simulink model "ElectricThrottleControl"  (R2024b)
settings: Solver=VariableStepAuto  StartTime=0.0  StopTime=0.5  RelTol=1e-3
settings Model: DataDictionary=SysMLArchModel_DD.sldd  Creator=ykamatan  LastModifiedBy=ykamatan
settings DataIOCC: ExternalInput=Scenario.getElement(1),Scenario.getElement(2),Scenario.getElement(3),Scenario.getElement(4)  LoadExternalInput=on

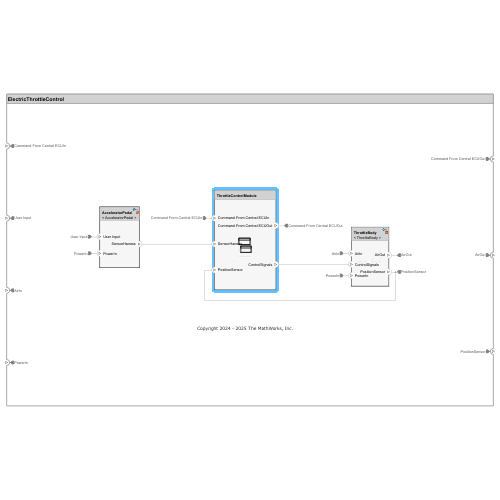
[thumbnail: Simulink's stored preview of the top-level diagram]
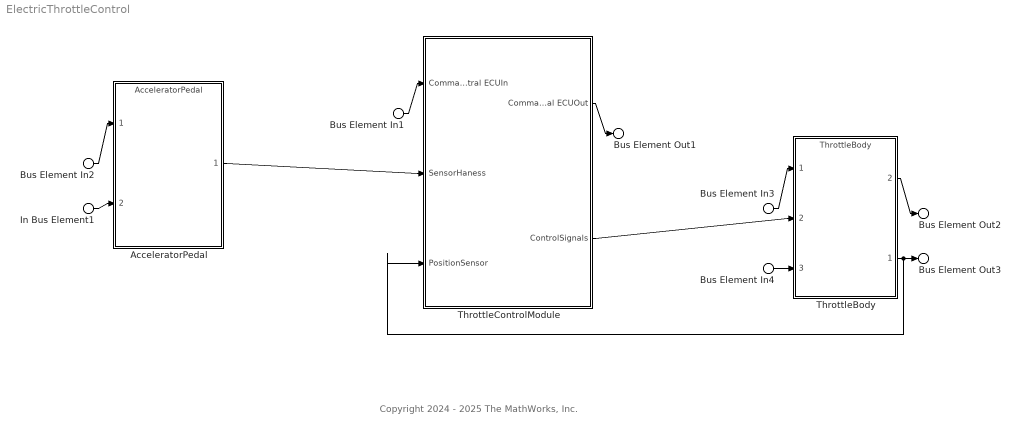
== system ElectricThrottleControl ==
  note: Copyright 2024 - 2025 The MathWorks, Inc.
  Bus Element In1 : Inport  PortName=Command From Central ECUIn
  Bus Element In2 : Inport  Port=2  PortName=User Input
  Bus Element In3 : Inport  Port=3  PortName=AirIn
  Bus Element In4 : Inport  Port=4  PortName=PowerIn
  In Bus Element1 : Inport  Port=4  PortName=PowerIn
  AcceleratorPedal : ModelReference  ModelNameDialog=AcceleratorPedal  SimulationMode=Normal  ModelReferenceVersion=1.6
      settings: PortSchema="{\"entries\":[{\"content\":{\"headerSize\":38,\"margin\":15,\"minimumSpacing\":25,\"sides\":[{\"content\":{\"connectorIds\":[\"In1\",\"In2\"]},\"type\":\"ConnectorPlacement.EquallySpacedRectSide\",\"uuid\":\"1abb2ddf-551e-4f22-91e6-e0600bbcfdfe\"},{\"content\":{\"connectorIds\":[\"Out1\"],\"side\":\"RIGHT\"},\"type\":\"ConnectorPlacement.EquallySpacedRectSide\",\"uuid\":\"67bebb00-cc4b-4347-b86c-01c9aefb7a18\"},{\"content\":{\"side\":\"TOP\"},\"type\":\"ConnectorPlacement.EquallySpacedRectSide\",\"uuid\":\"4c338e4e-b99e-491b-b4b2-5dc7867eebc8\"}]},\"type\":\"ConnectorPlacement.EquallySpacedConnector\",\"uuid\":\"67761126-1f2c-45f7-9918-87ef92113f7f\"}],\"packageUris\":[\"http://schema.mathworks.com/mf0/Connector/R2020b\"],\"version\":\"1.0\"}"
  ThrottleBody : ModelReference  ModelNameDialog=ThrottleBody  UsingDefaultArgumentValue=0,0,0,0,0,0,0  SimulationMode=Normal  ModelReferenceVersion=2.0
      settings: PortSchema="{\"entries\":[{\"content\":{\"headerSize\":38,\"margin\":15,\"minimumSpacing\":25,\"sides\":[{\"content\":{\"connectorIds\":[\"In1\",\"In2\",\"In3\"]},\"type\":\"ConnectorPlacement.EquallySpacedRectSide\",\"uuid\":\"1abb2ddf-551e-4f22-91e6-e0600bbcfdfe\"},{\"content\":{\"connectorIds\":[\"Out2\",\"Out1\"],\"side\":\"RIGHT\"},\"type\":\"ConnectorPlacement.EquallySpacedRectSide\",\"uuid\":\"67bebb00-cc4b-4347-b86c-01c9aefb7a18\"},{\"content\":{\"side\":\"TOP\"},\"type\":\"ConnectorPlacement.EquallySpacedRectSide\",\"uuid\":\"4c338e4e-b99e-491b-b4b2-5dc7867eebc8\"}]},\"type\":\"ConnectorPlacement.EquallySpacedConnector\",\"uuid\":\"67761126-1f2c-45f7-9918-87ef92113f7f\"}],\"packageUris\":[\"http://schema.mathworks.com/mf0/Connector/R2020b\"],\"version\":\"1.0\"}"
  ThrottleControlModule : Subsystem
      settings: PortSchema="{\"entries\":[{\"content\":{\"headerSize\":26,\"margin\":15,\"minimumSpacing\":25,\"sides\":[{\"content\":{\"connectorIds\":[\"In1\",\"In2\",\"In3\"]},\"type\":\"ConnectorPlacement.EquallySpacedRectSide\",\"uuid\":\"1abb2ddf-551e-4f22-91e6-e0600bbcfdfe\"},{\"content\":{\"connectorIds\":[\"Out1\",\"Out2\"],\"side\":\"RIGHT\"},\"type\":\"ConnectorPlacement.EquallySpacedRectSide\",\"uuid\":\"67bebb00-cc4b-4347-b86c-01c9aefb7a18\"},{\"content\":{\"side\":\"TOP\"},\"type\":\"ConnectorPlacement.EquallySpacedRectSide\",\"uuid\":\"4c338e4e-b99e-491b-b4b2-5dc7867eebc8\"}]},\"type\":\"ConnectorPlacement.EquallySpacedConnector\",\"uuid\":\"67761126-1f2c-45f7-9918-87ef92113f7f\"}],\"packageUris\":[\"http://schema.mathworks.com/mf0/Connector/R2020b\"],\"version\":\"1.0\"}"
  Bus Element Out1 : Outport  PortName=Command From Central ECUOut
  Bus Element Out2 : Outport  Port=2  PortName=AirOut
  Bus Element Out3 : Outport  Port=3  PortName=PositionSensor
  wires:
  Bus Element In1/1 -> ThrottleControlModule/1(Command From Central ECUIn)
  ThrottleControlModule/1(Command From Central ECUOut) -> Bus Element Out1/1
  In Bus Element1/1 -> AcceleratorPedal/2
  Bus Element In2/1 -> AcceleratorPedal/1
  AcceleratorPedal/1 -> ThrottleControlModule/2(SensorHaness)
  Bus Element In3/1 -> ThrottleBody/1
  ThrottleControlModule/2(ControlSignals) -> ThrottleBody/2
  Bus Element In4/1 -> ThrottleBody/3
  ThrottleBody/2 -> Bus Element Out2/1
  ThrottleBody/1 -> ThrottleControlModule/3(PositionSensor), Bus Element Out3/1

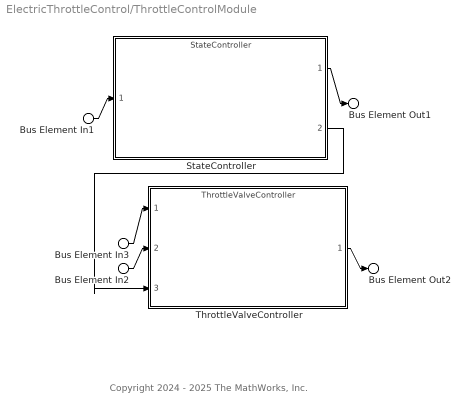
== system ElectricThrottleControl/ThrottleControlModule ==
  note: Copyright 2024 - 2025 The MathWorks, Inc.
  Bus Element In1 : Inport  PortName=Command From Central ECUIn
  Bus Element In2 : Inport  Port=2  PortName=SensorHaness
  Bus Element In3 : Inport  Port=3  PortName=PositionSensor
  StateController : ModelReference  ModelNameDialog=StateController  SimulationMode=Normal  ModelReferenceVersion=1.8
      settings: PortSchema="{\"entries\":[{\"content\":{\"headerSize\":38,\"margin\":15,\"minimumSpacing\":25,\"sides\":[{\"content\":{\"connectorIds\":[\"In1\"]},\"type\":\"ConnectorPlacement.EquallySpacedRectSide\",\"uuid\":\"1abb2ddf-551e-4f22-91e6-e0600bbcfdfe\"},{\"content\":{\"connectorIds\":[\"Out1\",\"Out2\"],\"side\":\"RIGHT\"},\"type\":\"ConnectorPlacement.EquallySpacedRectSide\",\"uuid\":\"67bebb00-cc4b-4347-b86c-01c9aefb7a18\"},{\"content\":{\"side\":\"TOP\"},\"type\":\"ConnectorPlacement.EquallySpacedRectSide\",\"uuid\":\"4c338e4e-b99e-491b-b4b2-5dc7867eebc8\"}]},\"type\":\"ConnectorPlacement.EquallySpacedConnector\",\"uuid\":\"67761126-1f2c-45f7-9918-87ef92113f7f\"}],\"packageUris\":[\"http://schema.mathworks.com/mf0/Connector/R2020b\"],\"version\":\"1.0\"}"
  ThrottleValveController : ModelReference  ModelNameDialog=ThrottleValveController  SimulationMode=Normal  ModelReferenceVersion=2.0
      settings: PortSchema="{\"entries\":[{\"content\":{\"headerSize\":38,\"margin\":15,\"minimumSpacing\":25,\"sides\":[{\"content\":{\"connectorIds\":[\"In1\",\"In2\",\"In3\"]},\"type\":\"ConnectorPlacement.EquallySpacedRectSide\",\"uuid\":\"1abb2ddf-551e-4f22-91e6-e0600bbcfdfe\"},{\"content\":{\"connectorIds\":[\"Out1\"],\"side\":\"RIGHT\"},\"type\":\"ConnectorPlacement.EquallySpacedRectSide\",\"uuid\":\"67bebb00-cc4b-4347-b86c-01c9aefb7a18\"},{\"content\":{\"side\":\"TOP\"},\"type\":\"ConnectorPlacement.EquallySpacedRectSide\",\"uuid\":\"4c338e4e-b99e-491b-b4b2-5dc7867eebc8\"}]},\"type\":\"ConnectorPlacement.EquallySpacedConnector\",\"uuid\":\"67761126-1f2c-45f7-9918-87ef92113f7f\"}],\"packageUris\":[\"http://schema.mathworks.com/mf0/Connector/R2020b\"],\"version\":\"1.0\"}"
  Bus Element Out1 : Outport  PortName=Command From Central ECUOut
  Bus Element Out2 : Outport  Port=2  PortName=ControlSignals
  wires:
  Bus Element In1/1 -> StateController/1
  StateController/1 -> Bus Element Out1/1
  Bus Element In3/1 -> ThrottleValveController/1
  StateController/2 -> ThrottleValveController/3
  Bus Element In2/1 -> ThrottleValveController/2
  ThrottleValveController/1 -> Bus Element Out2/1
